simulink model "HandControl"  (R2024a)
settings: Solver=FixedStepDiscrete  StartTime=0.0  StopTime=10  FixedStep=0.01  RelTol=1e-3
PreLoadFcn:
  | if exist('HandControl_types', 'file') == 2, HandControl_types(); end
model workspace (MAT data in the model file):
  CoarseStep_mV = Simulink.Parameter
  CoarseStep_mV.Value = 15
  CoarseStep_mV.Complexity = 'real'
  CoarseStep_mV.Dimensions = [1 1]
  CoarseStep_mV.DataType = 'single'
  CountsPerStep = Simulink.Parameter
  CountsPerStep.Value = 4
  CountsPerStep.Complexity = 'real'
  CountsPerStep.Dimensions = [1 1]
  CountsPerStep.DataType = 'uint8'
  DisplayFilter_cycles = Simulink.Parameter
  DisplayFilter_cycles.Value = 30
  DisplayFilter_cycles.Complexity = 'real'
  DisplayFilter_cycles.Dimensions = [1 1]
  DisplayFilter_cycles.DataType = 'uint16'
  DisplayHyst_mV = Simulink.Parameter
  DisplayHyst_mV.Value = 3
  DisplayHyst_mV.Complexity = 'real'
  DisplayHyst_mV.Dimensions = [1 1]
  DisplayHyst_mV.DataType = 'uint16'
  DisplayJump_mV = Simulink.Parameter
  DisplayJump_mV.Value = 20
  DisplayJump_mV.Complexity = 'real'
  DisplayJump_mV.Dimensions = [1 1]
  DisplayJump_mV.DataType = 'uint16'
  FineStep_mV = Simulink.Parameter
  FineStep_mV.Value = 1
  FineStep_mV.Complexity = 'real'
  FineStep_mV.Dimensions = [1 1]
  FineStep_mV.DataType = 'single'
  HandMinSetpoint_V = Simulink.Parameter
  HandMinSetpoint_V.Value = 0.7
  HandMinSetpoint_V.Complexity = 'real'
  HandMinSetpoint_V.Dimensions = [1 1]
  HandMinSetpoint_V.DataType = 'single'
  KeyDebounce_cycles = Simulink.Parameter
  KeyDebounce_cycles.Value = 3
  KeyDebounce_cycles.Complexity = 'real'
  KeyDebounce_cycles.Dimensions = [1 1]
  KeyDebounce_cycles.DataType = 'uint8'
  SetpointLimit_V = Simulink.Parameter
  SetpointLimit_V.Value = 5
  SetpointLimit_V.Complexity = 'real'
  SetpointLimit_V.Dimensions = [1 1]
  SetpointLimit_V.DataType = 'single'
values from neighbouring files (symbols this model uses):
  CoarseStep_mV = 15    [HandControl_data.m]
  CountsPerStep = 4    [HandControl_data.m]
  DisplayFilter_cycles = 30    [HandControl_data.m]
  DisplayHyst_mV = 3    [HandControl_data.m]
  DisplayJump_mV = 20    [HandControl_data.m]
  FineStep_mV = 1    [HandControl_data.m]
  HandMinSetpoint_V = 0.7    [HandControl_data.m]
  KeyDebounce_cycles = 3    [HandControl_data.m]
  SetpointLimit_V = 5.0    (= 5)    [HandControl_data.m]
Description:
  | Handbetrieb: Drehgeber und Karten-Tasten zu Sollwerten und Freigaben der Kanaele, Kanalwahl, Anzeigewert
settings Model: ParameterArgumentNames=SetpointLimit_V,CoarseStep_mV,FineStep_mV,CountsPerStep,KeyDebounce_cycles,HandMinSetpoint_V,DisplayFilter_cycles,DisplayHyst_mV,DisplayJump_mV  Creator=danie  LastModifiedBy=danie
settings OptimizationCC: DefaultParameterBehavior=Inlined  EnhancedBackFolding=on  PassReuseOutputArgsAs=Individual arguments  ZeroExternalMemoryAtStartup=off  ZeroInternalMemoryAtStartup=off  OptimizeBlockOrder=speed  DifferentSizesBufferReuse=on  OptimizationCustomize=off  EfficientTunableParamExpr=on
settings DebuggingCC: ParameterTunabilityLossMsg=error
settings HardwareCC: ProdBitPerPointer=32  ProdBitPerSizeT=32  ProdBitPerPtrDiffT=32  ProdLargestAtomicInteger=Long  ProdLargestAtomicFloat=Double  ProdWordSize=32  ProdLongLongMode=on  ProdHWDeviceType=ARM Compatible->ARM Cortex-M
settings SFSimCC: MATLABDynamicMemAlloc=off
settings RTWCC: Description=AUTOSAR  SystemTargetFile=autosar.tlc  GenCodeOnly=on  GenerateMakefile=off  TemplateMakefile=ert_default_tmf  DataTypeReplacement=CDataTypesFixedWidth
settings CodeAppCC: ForceParamTrailComments=on  IgnoreCustomStorageClasses=off  MaxIdLength=63  OperatorAnnotations=on  SimulinkDataObjDesc=on  SFDataObjDesc=on  InsertBlockDesc=on
settings STFCustomTargetCC: MultiwordLength=256  ParMdlRefBuildCompliant=on  CompOptLevelCompliant=on  IncludeMdlTerminateFcn=off  CombineOutputUpdateFcns=on  SuppressErrorStatus=on  ERTCustomFileBanners=on  SupportNonFinite=off  SupportComplex=off  SupportContinuousTime=off  SupportNonInlinedSFcns=off  RemoveResetFunc=on  MATLABClassNameForMDSCustomization=Simulink.SoftwareTarget.ERTCustomization  AutosarCompliant=on  GRTInterface=off  LookupTableObjectStructAxisOrder=2,1,3,4,...  LUTObjectStructOrderEvenSpacing=Size,Table,Breakpoints  SystemTargetFile=autosar.tlc
settings ERTTargetCC: TargetLangStandard=C99 (ISO)  ConcurrentExecutionCompliant=off  IncludeMdlTerminateFcn=off  SuppressErrorStatus=on  SupportNonFinite=off  SupportComplex=off  ModelStepFunctionPrototypeControlCompliant=off  CPPClassGenCompliant=off  AutosarCompliant=on  LookupTableObjectStructAxisOrder=2,1,3,4,...  LUTObjectStructOrderEvenSpacing=Size,Table,Breakpoints  InlinedParameterPlacement=NonHierarchical  ERTCustomFileTemplate=example_file_process.tlc  BooleanTrueId=TRUE  BooleanFalseId=FALSE

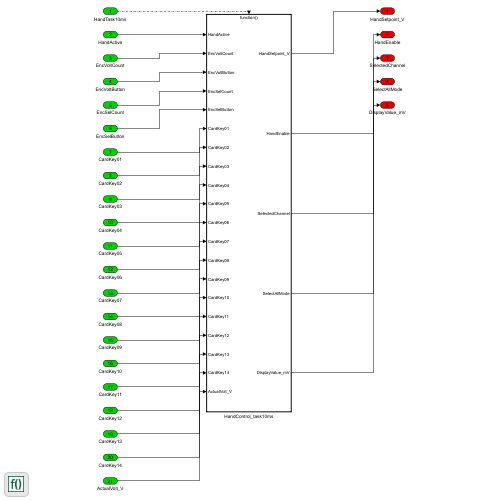
[thumbnail: Simulink's stored preview of the top-level diagram]
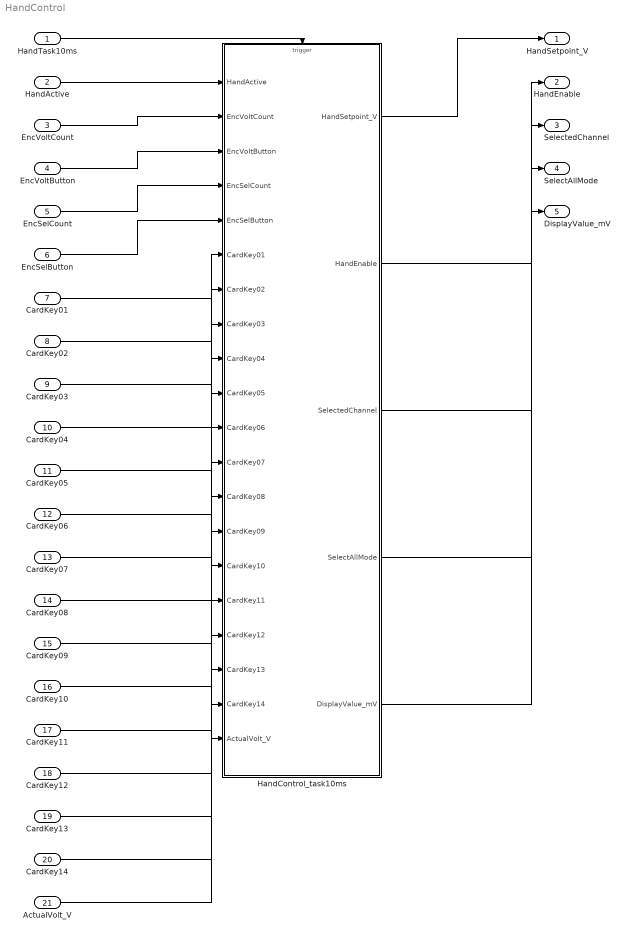
== system HandControl ==
  HandTask10ms : Inport  SampleTime=0.01  OutputFunctionCall=on
  HandActive : Inport  Port=2  OutDataTypeStr=boolean  PortDimensions=1
  EncVoltCount : Inport  Port=3  OutDataTypeStr=uint16  PortDimensions=1
  EncVoltButton : Inport  Port=4  OutDataTypeStr=boolean  PortDimensions=1
  EncSelCount : Inport  Port=5  OutDataTypeStr=uint16  PortDimensions=1
  EncSelButton : Inport  Port=6  OutDataTypeStr=boolean  PortDimensions=1
  CardKey01 : Inport  Port=7  OutDataTypeStr=boolean  PortDimensions=1
  CardKey02 : Inport  Port=8  OutDataTypeStr=boolean  PortDimensions=1
  CardKey03 : Inport  Port=9  OutDataTypeStr=boolean  PortDimensions=1
  CardKey04 : Inport  Port=10  OutDataTypeStr=boolean  PortDimensions=1
  CardKey05 : Inport  Port=11  OutDataTypeStr=boolean  PortDimensions=1
  CardKey06 : Inport  Port=12  OutDataTypeStr=boolean  PortDimensions=1
  CardKey07 : Inport  Port=13  OutDataTypeStr=boolean  PortDimensions=1
  CardKey08 : Inport  Port=14  OutDataTypeStr=boolean  PortDimensions=1
  CardKey09 : Inport  Port=15  OutDataTypeStr=boolean  PortDimensions=1
  CardKey10 : Inport  Port=16  OutDataTypeStr=boolean  PortDimensions=1
  CardKey11 : Inport  Port=17  OutDataTypeStr=boolean  PortDimensions=1
  CardKey12 : Inport  Port=18  OutDataTypeStr=boolean  PortDimensions=1
  CardKey13 : Inport  Port=19  OutDataTypeStr=boolean  PortDimensions=1
  CardKey14 : Inport  Port=20  OutDataTypeStr=boolean  PortDimensions=1
  ActualVolt_V : Inport  Port=21  OutDataTypeStr=single  PortDimensions=CellCount
  HandControl_task10ms : Subsystem  TreatAsAtomicUnit=on
  HandSetpoint_V : Outport  OutDataTypeStr=single  PortDimensions=CellCount
  HandEnable : Outport  Port=2  OutDataTypeStr=boolean  PortDimensions=CellCount
  SelectedChannel : Outport  Port=3  OutDataTypeStr=uint8  PortDimensions=1
  SelectAllMode : Outport  Port=4  OutDataTypeStr=boolean  PortDimensions=1
  DisplayValue_mV : Outport  Port=5  OutDataTypeStr=uint16  PortDimensions=1
  wires:
  HandTask10ms/1 -> HandControl_task10ms/Trigger
  HandActive/1 -> HandControl_task10ms/1(HandActive)
  EncVoltCount/1 -> HandControl_task10ms/2(EncVoltCount)
  EncVoltButton/1 -> HandControl_task10ms/3(EncVoltButton)
  EncSelCount/1 -> HandControl_task10ms/4(EncSelCount)
  EncSelButton/1 -> HandControl_task10ms/5(EncSelButton)
  CardKey01/1 -> HandControl_task10ms/6(CardKey01)
  CardKey02/1 -> HandControl_task10ms/7(CardKey02)
  CardKey03/1 -> HandControl_task10ms/8(CardKey03)
  CardKey04/1 -> HandControl_task10ms/9(CardKey04)
  CardKey05/1 -> HandControl_task10ms/10(CardKey05)
  CardKey06/1 -> HandControl_task10ms/11(CardKey06)
  CardKey07/1 -> HandControl_task10ms/12(CardKey07)
  CardKey08/1 -> HandControl_task10ms/13(CardKey08)
  CardKey09/1 -> HandControl_task10ms/14(CardKey09)
  CardKey10/1 -> HandControl_task10ms/15(CardKey10)
  CardKey11/1 -> HandControl_task10ms/16(CardKey11)
  CardKey12/1 -> HandControl_task10ms/17(CardKey12)
  CardKey13/1 -> HandControl_task10ms/18(CardKey13)
  CardKey14/1 -> HandControl_task10ms/19(CardKey14)
  ActualVolt_V/1 -> HandControl_task10ms/20(ActualVolt_V)
  HandControl_task10ms/1(HandSetpoint_V) -> HandSetpoint_V/1
  HandControl_task10ms/2(HandEnable) -> HandEnable/1
  HandControl_task10ms/3(SelectedChannel) -> SelectedChannel/1
  HandControl_task10ms/4(SelectAllMode) -> SelectAllMode/1
  HandControl_task10ms/5(DisplayValue_mV) -> DisplayValue_mV/1

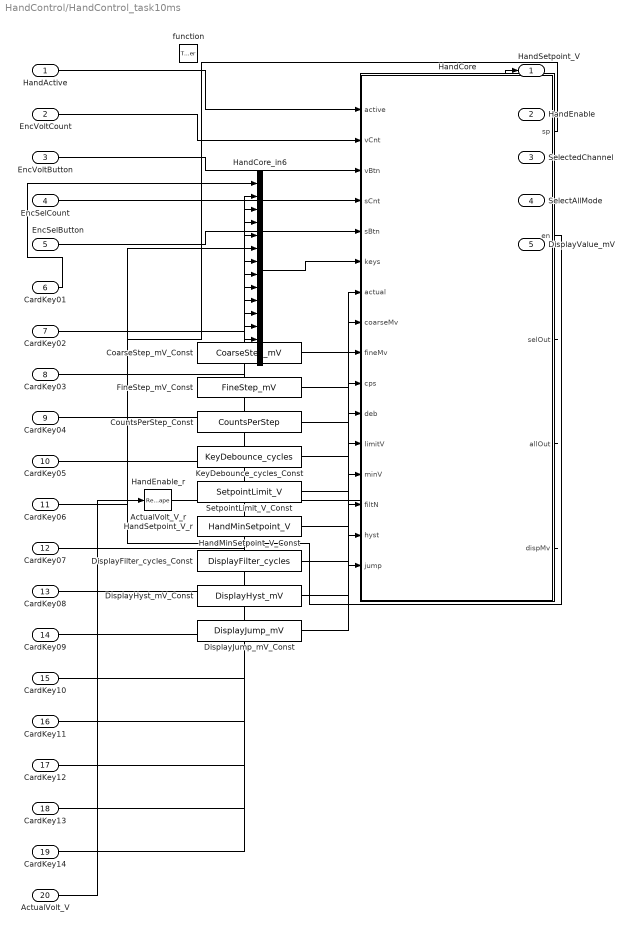
== system HandControl/HandControl_task10ms ==
  HandActive : Inport
  EncVoltCount : Inport  Port=2
  EncVoltButton : Inport  Port=3
  EncSelCount : Inport  Port=4
  EncSelButton : Inport  Port=5
  CardKey01 : Inport  Port=6
  CardKey02 : Inport  Port=7
  CardKey03 : Inport  Port=8
  CardKey04 : Inport  Port=9
  CardKey05 : Inport  Port=10
  CardKey06 : Inport  Port=11
  CardKey07 : Inport  Port=12
  CardKey08 : Inport  Port=13
  CardKey09 : Inport  Port=14
  CardKey10 : Inport  Port=15
  CardKey11 : Inport  Port=16
  CardKey12 : Inport  Port=17
  CardKey13 : Inport  Port=18
  CardKey14 : Inport  Port=19
  ActualVolt_V : Inport  Port=20
  function : TriggerPort  TriggerType=function-call  VariantControl=(inherit)  SampleTimeType=periodic  SampleTime=0.01
  ActualVolt_V_r : Reshape  OutputDimensionality=Customize  OutputDimensions=[14 1]
  CoarseStep_mV_Const : Constant  Value=CoarseStep_mV  OutDataTypeStr=single
  CountsPerStep_Const : Constant  Value=CountsPerStep  OutDataTypeStr=uint8
  DisplayFilter_cycles_Const : Constant  Value=DisplayFilter_cycles  OutDataTypeStr=uint16
  DisplayHyst_mV_Const : Constant  Value=DisplayHyst_mV  OutDataTypeStr=uint16
  DisplayJump_mV_Const : Constant  Value=DisplayJump_mV  OutDataTypeStr=uint16
  FineStep_mV_Const : Constant  Value=FineStep_mV  OutDataTypeStr=single
  HandCore : MATLAB Function  TreatAsAtomicUnit=on
  HandCore_in6 : Mux  Inputs=14
  HandEnable_r : Reshape
  HandMinSetpoint_V_Const : Constant  Value=HandMinSetpoint_V  OutDataTypeStr=single
  HandSetpoint_V_r : Reshape
  KeyDebounce_cycles_Const : Constant  Value=KeyDebounce_cycles  OutDataTypeStr=uint8
  SetpointLimit_V_Const : Constant  Value=SetpointLimit_V  OutDataTypeStr=single
  HandSetpoint_V : Outport
  HandEnable : Outport  Port=2
  SelectedChannel : Outport  Port=3
  SelectAllMode : Outport  Port=4
  DisplayValue_mV : Outport  Port=5
  wires:
  ActualVolt_V/1 -> ActualVolt_V_r/1
  HandSetpoint_V_r/1 -> HandSetpoint_V/1
  HandEnable_r/1 -> HandEnable/1
  HandActive/1 -> HandCore/1(active)
  EncVoltCount/1 -> HandCore/2(vCnt)
  EncVoltButton/1 -> HandCore/3(vBtn)
  EncSelCount/1 -> HandCore/4(sCnt)
  EncSelButton/1 -> HandCore/5(sBtn)
  CardKey01/1 -> HandCore_in6/1
  CardKey02/1 -> HandCore_in6/2
  CardKey03/1 -> HandCore_in6/3
  CardKey04/1 -> HandCore_in6/4
  CardKey05/1 -> HandCore_in6/5
  CardKey06/1 -> HandCore_in6/6
  CardKey07/1 -> HandCore_in6/7
  CardKey08/1 -> HandCore_in6/8
  CardKey09/1 -> HandCore_in6/9
  CardKey10/1 -> HandCore_in6/10
  CardKey11/1 -> HandCore_in6/11
  CardKey12/1 -> HandCore_in6/12
  CardKey13/1 -> HandCore_in6/13
  CardKey14/1 -> HandCore_in6/14
  HandCore_in6/1 -> HandCore/6(keys)
  ActualVolt_V_r/1 -> HandCore/7(actual)
  CoarseStep_mV_Const/1 -> HandCore/8(coarseMv)
  FineStep_mV_Const/1 -> HandCore/9(fineMv)
  CountsPerStep_Const/1 -> HandCore/10(cps)
  KeyDebounce_cycles_Const/1 -> HandCore/11(deb)
  SetpointLimit_V_Const/1 -> HandCore/12(limitV)
  HandMinSetpoint_V_Const/1 -> HandCore/13(minV)
  DisplayFilter_cycles_Const/1 -> HandCore/14(filtN)
  DisplayHyst_mV_Const/1 -> HandCore/15(hyst)
  DisplayJump_mV_Const/1 -> HandCore/16(jump)
  HandCore/1(sp) -> HandSetpoint_V_r/1
  HandCore/2(en) -> HandEnable_r/1
  HandCore/3(selOut) -> SelectedChannel/1
  HandCore/4(allOut) -> SelectAllMode/1
  HandCore/5(dispMv) -> DisplayValue_mV/1

== matlab function HandControl/HandControl_task10ms/HandCore ==
  data: active input; sp output; vCnt input; vBtn input; sCnt input; sBtn input; keys input; actual input; coarseMv input; fineMv input; cps input; deb input; limitV input; minV input; filtN input; hyst input; jump input; en output; selOut output; allOut output; dispMv output
function [sp, en, selOut, allOut, dispMv] = HandCore(active, vCnt, vBtn, sCnt, sBtn, keys, actual, coarseMv, fineMv, cps, deb, limitV, minV, filtN, hyst, jump)
%HANDCORE Hand mode: encoders, keys, setpoints, releases, selection and display value (see HandControl_create.m).
%#codegen
persistent started lastV lastS accV accS sel coarse selAll spMv en0 wasActive cntV cntS cntK filt shown lastSel dispInit
if isempty(started)
    started = true;
    lastV = vCnt;
    lastS = sCnt;
    accV = int32(0);
    accS = int32(0);
    sel = uint8(1);
    coarse = true;
    selAll = false;
    spMv = zeros(14, 1, 'int32');
    en0 = false(14, 1);
    wasActive = false;
    cntV = uint8(0);
    cntS = uint8(0);
    cntK = zeros(14, 1, 'uint8');
    filt = single(0);
    shown = single(0);
    lastSel = uint8(1);
    dispInit = false;
end
debounce = max(deb, uint8(1));
% encoders: counter difference with the wrap of the 16 bit counter, whole detents
accV = accV + wrapDiff(vCnt, lastV);
accS = accS + wrapDiff(sCnt, lastS);
lastV = vCnt;
lastS = sCnt;
perStep = int32(max(cps, uint8(1)));
stepsV = int32(0);
stepsS = int32(0);
if abs(accV) >= perStep
    stepsV = idivide(accV, perStep, 'fix');
    accV = accV - stepsV * perStep;
end
if abs(accS) >= perStep
    stepsS = idivide(accS, perStep, 'fix');
    accS = accS - stepsS * perStep;
end
% keys: one event per press, after the debounce time
[cntV, evV] = pressed(vBtn, cntV, debounce);
[cntS, evS] = pressed(sBtn, cntS, debounce);
evK = false(14, 1);
for k = 1:14
    [cntK(k), evK(k)] = pressed(keys(k), cntK(k), debounce);
end
if evV
    coarse = ~coarse;
end
if evS
    selAll = ~selAll;
end
% channel selection, saturating
newSel = int32(sel) + stepsS;
if newSel < int32(1)
    newSel = int32(1);
elseif newSel > int32(14)
    newSel = int32(14);
end
sel = uint8(newSel);
limitMv = int32(round(limitV * single(1000)));
if active
    if ~wasActive
        spMv = zeros(14, 1, 'int32');
        en0 = true(14, 1);
    end
    if stepsV ~= int32(0)
        if coarse
            stepMv = coarseMv;
        else
            stepMv = fineMv;
        end
        v = spMv(sel) + int32(round(single(stepsV) * stepMv));
        minMv = int32(round(minV * single(1000)));
        if (v > int32(0)) && (v < minMv)       % the gap 0 .. minimum is jumped over, up to the minimum or down to 0
            if stepsV > int32(0)
                v = minMv;
            else
                v = int32(0);
            end
        end
        if v < int32(0)
            v = int32(0);
        elseif v > limitMv
            v = limitMv;
        end
        if selAll
            spMv = v * ones(14, 1, 'int32');
        else
            spMv(sel) = v;
        end
    end
    for k = 1:14
        if evK(k)
            en0(k) = ~en0(k);
        end
    end
else
    spMv = zeros(14, 1, 'int32');
    en0 = false(14, 1);
end
wasActive = active;
sp = single(spMv) / single(1000);
en = en0;
selOut = sel;
allOut = selAll;
x = actual(sel) * single(1000);
% written so that a value that is not a number ends in the last branch (0), also after the optimisation of the code generator
y = single(0);
if x > single(9999)
    y = single(9999);
elseif x >= single(0)
    y = x;
end
% display: new channel or a large deviation at once, otherwise PT1 and a hysteresis on the shown value
n = single(max(filtN, uint16(1)));
if (~dispInit) || (sel ~= lastSel) || (abs(y - filt) >= single(jump))
    filt = y;
    shown = round(y);
else
    filt = filt + (y - filt) / n;
    if abs(filt - shown) >= single(hyst)
        shown = round(filt);
    end
end
lastSel = sel;
dispInit = true;
dispMv = uint16(shown);

function d = wrapDiff(cur, prev)
% difference of two readings of a 16 bit counter, -32768 .. 32767
d = int32(cur) - int32(prev);
if d > int32(32767)
    d = d - int32(65536);
elseif d < int32(-32768)
    d = d + int32(65536);
end

function [cnt, ev] = pressed(down, cnt, debounce)
ev = false;
if down
    if cnt < uint8(255)
        cnt = cnt + uint8(1);
        if cnt == debounce
            ev = true;
        end
    end
else
    cnt = uint8(0);
end
